simulink library "Pitch_Actuation_Linkage_Lib"  (R2025a)
settings: Solver=ode45  StartTime=0.0  StopTime=10.0  RelTol=1e-3  EnableMultiTasking=on
Description:
  | Copyright 2009-2025 The MathWorks, Inc. MathWorks, Inc.
settings Model: Creator=smiller  LastModifiedBy=smiller
settings SolverCC: AlgebraicLoopSolver=TrustRegion
settings DataIOCC: LimitDataPoints=on  SaveFormat=Array  SignalLoggingSaveFormat=ModelDataLogs  ReturnWorkspaceOutputs=off
settings OptimizationCC: ReuseModelBlockBuffer=off  ExpressionDepthLimit=2147483647.0  LifeSpan=inf
settings DebuggingCC: UnderspecifiedInitializationDetection=Classic  MergeDetectMultiDrivingBlocksExec=none  SolverPrmCheckMsg=warning  FcnCallInpInsideContextMsg=warning  UnconnectedInputMsg=warning  UnconnectedOutputMsg=warning  UnconnectedLineMsg=warning  AllowSymbolicDim=off  StateNameClashWarn=warning  PregeneratedLibrarySubsystemCodeDiagnostic=none  SFUnexpectedBacktrackingDiag=warning  SFNoUnconditionalDefaultTransitionDiag=warning  SFExecutionAtInitializationDiag=none  ArithmeticOperatorsInVariantConditions=warning
settings HardwareCC: ProdBitPerPointer=32.0  ProdBitPerSizeT=32.0  ProdBitPerPtrDiffT=32.0  ProdLargestAtomicFloat=None  ProdIntDivRoundTo=Undefined  ProdEndianess=Unspecified  ProdWordSize=32.0  ProdHWDeviceType=32-bit Generic
settings ModelReferenceCC: EnableRefExpFcnMdlSchedulingChecks=on  PropagateSignalLabelsOutOfModel=off
settings SFSimCC: SimUseLocalCustomCode=off  CustomCodeUndefinedFunction=UseInterfaceOnly
settings RTWCC: RTWUseLocalCustomCode=off  GPUComputeCapability=3.5  DLArmComputeVersion=19.05
settings CodeAppCC: StateflowObjectComments=on
settings GRTTargetCC: TargetLangStandard=C89/C90 (ANSI)  CombineOutputUpdateFcns=off  GRTInterface=on
settings ConfigComp: CovMetricSettings=dw  CovSaveCumulativeToWorkspaceVar=on  CovSaveSingleToWorkspaceVar=on  CovExternalEMLEnable=off  CovSFcnEnable=off

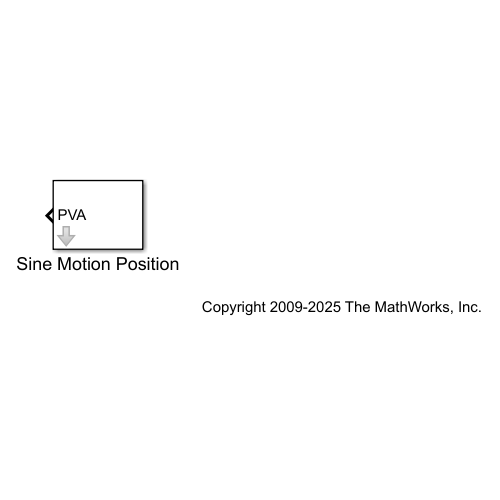
[thumbnail: Simulink's stored preview of the top-level diagram]
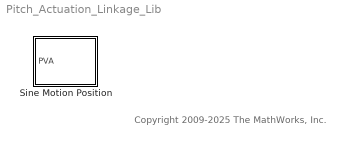
== system Pitch_Actuation_Linkage_Lib ==
  note: Copyright 2009-2025 The MathWorks, Inc.
  Sine Motion Position : Subsystem  mask{Amplitude=0.2, pd=5, PhaseShift=0}
      mask prompts: pd "Period (Seconds)"; PhaseShift "Phase Shift (Degrees)"

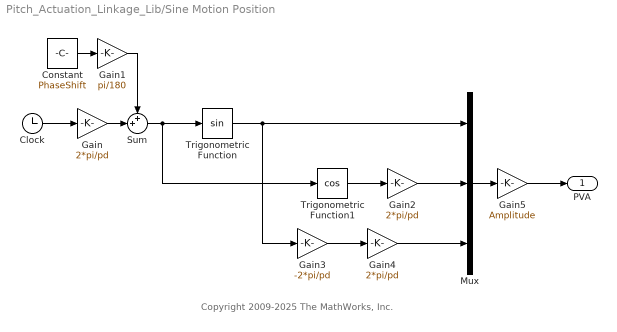
== system Pitch_Actuation_Linkage_Lib/Sine Motion Position ==
  note: Copyright 2009-2025 The MathWorks, Inc.
  Clock : Clock
  Constant : Constant  Value=PhaseShift
  Gain : Gain  Gain=2*pi/pd
  Gain1 : Gain  Gain=pi/180
  Gain2 : Gain  Gain=2*pi/pd
  Gain3 : Gain  Gain=-2*pi/pd
  Gain4 : Gain  Gain=2*pi/pd
  Gain5 : Gain  Gain=Amplitude
  Mux : Mux  Inputs=3
  Sum : Sum  Inputs=++|
  Trigonometric Function : Trigonometry
  Trigonometric Function1 : Trigonometry  Operator=cos
  PVA : Outport  VectorParamsAs1DForOutWhenUnconnected=off
  wires:
  Gain4/1 -> Mux/3
  Gain3/1 -> Gain4/1
  Gain2/1 -> Mux/2
  Trigonometric Function1/1 -> Gain2/1
  Gain5/1 -> PVA/1
  Mux/1 -> Gain5/1
  Trigonometric Function/1 -> Gain3/1, Mux/1
  Sum/1 -> Trigonometric Function1/1, Trigonometric Function/1
  Gain1/1 -> Sum/1
  Constant/1 -> Gain1/1
  Gain/1 -> Sum/2
  Clock/1 -> Gain/1
